simulink model "mppt_solar"  (R2024b)
settings: Solver=VariableStepAuto  StartTime=0.0  StopTime=1  RelTol=1e-3
libraries: spsSeriesRLCBranchLib x4, spsDiodeLib x2, spsCurrentMeasurementLib x1, spsMosfetLib x1, spsPVArrayLib x1, spsPWMGeneratorDCDCLib x1, spsVoltageMeasurementLib x1, spspowerguiLib x1
settings Model: Creator=saaka  LastModifiedBy=Ram
settings ModelReferenceCC: EnableRefExpFcnMdlSchedulingChecks=on
settings RTWCC: GPUComputeCapability=3.5

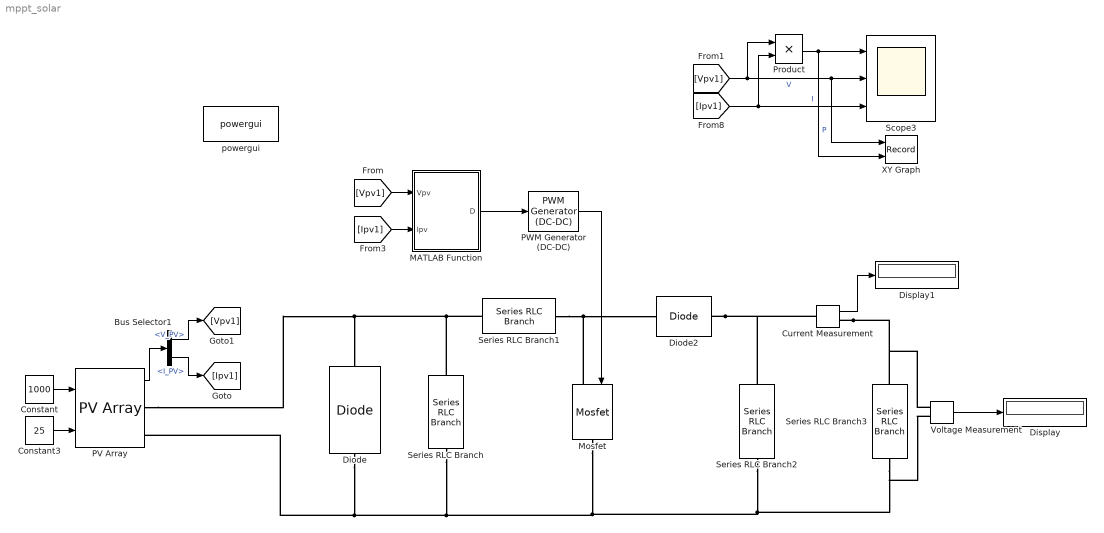
== system mppt_solar ==
  Bus Selector1 : BusSelector  OutputSignals=V_PV,I_PV
  Constant : Constant  Value=1000
  Constant3 : Constant  Value=25
  Current Measurement : spsCurrentMeasurementLib/Current Measurement  PhasorSimulation=off  OutputType=Complex  PSBequivalent=0
  Diode : spsDiodeLib/Diode  Ron=0.001  Lon=0  Vf=0.8  IC=0  UseSnubber=0  Rs=500  Cs=250e-9  Measurements=off
  Diode2 : spsDiodeLib/Diode  Ron=0.001  Lon=0  Vf=0.8  IC=0  UseSnubber=0  Rs=500  Cs=250e-9  Measurements=off
  Display : Display
  Display1 : Display
  MATLAB Function : MATLAB Function  TreatAsAtomicUnit=on
  Mosfet : spsMosfetLib/Mosfet  Ron=0.1  Lon=0  Rd=0.01  Vfd=0  IC=0  Rs=1e5  Cs=inf  Measurements=off
  PV Array : spsPVArrayLib/PV Array  Npar=1  Nser=1  PlotType=array @ 1000 W/m2 & specified temperatures  S_vec="[ 1000  500  100 ]"  Temp_C_vec="[ 45 25  ]"  ModuleName=User-defined  PlotWhenSelected=off  Pm=40.04  Ncell=36  Voc=22.5  Isc=2.22  Vm=19.25  Im=2.08  beta_Voc_pc=-0.36099  alpha_Isc_pc=0.102  beta_Voc=-0.081223  alpha_Isc=0.0022644  IL=2.2218  I0=8.2538e-11  nI=1.0138  Rsh=483.6839  Rs=0.18035  RobustModel=off  RobustCellTemperature=313.3991  BAL=on  Tc=1e-6  Tfilter=5e-5
  PWM Generator (DC-DC) : spsPWMGeneratorDCDCLib/PWM Generator (DC-DC)  Fsw=5000  Ts=0
  Product : Product
  Scope3 : Scope  NumInputPorts=3
  Series RLC Branch : spsSeriesRLCBranchLib/Series RLC Branch  LConnTagsString=__new0  RConnTagsString=__new0  BranchType=C  Resistance=1  Inductance=1e-3  SetiL0=off  InitialCurrent=0  Capacitance=300e-6  Setx0=off  InitialVoltage=0  Measurements=None
  Series RLC Branch1 : spsSeriesRLCBranchLib/Series RLC Branch  LConnTagsString=__new0  RConnTagsString=__new0  BranchType=L  Resistance=1  Inductance=2e-3  SetiL0=off  InitialCurrent=0  Capacitance=1e-6  Setx0=off  InitialVoltage=0  Measurements=None
  Series RLC Branch2 : spsSeriesRLCBranchLib/Series RLC Branch  LConnTagsString=__new0  RConnTagsString=__new0  BranchType=C  Resistance=1  Inductance=1e-3  SetiL0=off  InitialCurrent=0  Capacitance=220e-6  Setx0=off  InitialVoltage=0  Measurements=None
  Series RLC Branch3 : spsSeriesRLCBranchLib/Series RLC Branch  LConnTagsString=__new0  RConnTagsString=__new0  BranchType=R  Resistance=20  Inductance=1e-3  SetiL0=off  InitialCurrent=0  Capacitance=1e-6  Setx0=off  InitialVoltage=0  Measurements=None
  Voltage Measurement : spsVoltageMeasurementLib/Voltage Measurement  PhasorSimulation=off  OutputType=Complex  PSBequivalent=0
  XY Graph : Record  FileSettingsInternal="{\"entries\":[{\"content\":{\"excelSettings\":{\"content\":{},\"type\":\"Streamout.ExcelSettings\"}},\"type\":\"Streamout.FileSettingStorage\",\"uuid\":\"\"}],\"packageUris\":[\"http:\\/\\/schema.mathworks.com\\/mf0\\/streamout_blocks\\/R2020a\"],\"version\":\"1.0\"}"  Layout=[1 1]  SignalsInternal="{\"entries\":[{\"content\":{\"signals\":[{\"content\":{\"blockPath\":[],\"dimensions\":[1],\"domain\":\"\",\"lineColor\":\"#a2142f\",\"plots\":[ 1 ],\"port\":1,\"sid\":[\"\"],\"signalID\":1,\"signalName\":\"V\"},\"type\":\"RecordBlkView.Signal\",\"uuid\":\"\"},{\"content\":{\"blockPath\":[],\"dimensions\":[1],\"domain\":\"\",\"lineColor\":\"#139fff\",\"plots\":[ 1 ],\"port\":2,\"sid\":[\"\"],\"signalID\":2,\"signalName\":\"P\"},\"type\":\"RecordBlkView.Signal\",\"uuid\":\"\"}]},\"type\":\"RecordBlkView.InputSignals\",\"uuid\":\"\"}],\"packageUris\":[\"http:\\/\\/schema.mathworks.com\\/mf0\\/streamout_blocks\\/R2020a\"],\"version\":\"1.0\"}"  VisualizationBindings="{\"xyplotplugin\":{\"info\":[{\"series\":[{\"bindingParametersList\":[{\"parameter\":\"X-Axis\",\"signalID\":1,\"signalName\":\"V\"},{\"parameter\":\"Y-Axis\",\"signalID\":2,\"signalName\":\"P\"},{\"parameter\":\"X-Axis\",\"signalID\":1,\"signalName\":\"V\"},{\"parameter\":\"Y-Axis\",\"signalID\":2,\"signalName\":\"P\"}],\"seriesID\":0}],\"subplotID\":1}]}}"  CompatibilityTag=XY
  powergui : spspowerguiLib/powergui  Priority=1  SimulationMode=Continuous  SampleTime=50e-6  frequency=60  Iterations=50  frequencyindice=0  Pbase=100e6  ErrMax=1e-4  UnitsV=kV  UnitsW=MW  buscounter=0  FunctionMessages=off  echomessages=off  EnableUseOfTLC=off  CurrentSourceSwitches=off  DisableSnubberDevices=off  DisableRonSwitches=off  DisableVfSwitches=off  DisplayEquations=off  AutomaticDiscreteSolvers=off  SolverType=Tustin/Backward Euler (TBE)  Interpol=off  ExternalGateDelay=off  methode=off  Ts=100  x0status=blocks  SPID=on  SwTol=0  HookPort=off  NonlinearTolerance=1e-4  nMaxIteration=100  ContinueOnMaxIteration=off  RestoreLinks=warning  ResistiveCurrentMeasurement=off  Frange=[0:2:500]  Ylog=off  Xlog=on  ShowGrid=off  save=off  variable=ZData  structure=0  ZoomFFT=off  StartTime=0.0  cycles=1  DisplayStyle=1  fundamental=60  FreqAxis=off  MaxFrequency=1000  frequencyindicesteady=1  RmsSteady=1  display=off
  wires:
  Constant/1 -> PV Array/1
  Constant3/1 -> PV Array/2
  Current Measurement/1 -> Display1/1
  Voltage Measurement/1 -> Display/1
  [Vpv1] -> MATLAB Function/1(Vpv)
  [Ipv1] -> MATLAB Function/2(Ipv)
  MATLAB Function/1(D) -> PWM Generator (DC-DC)/1
  PWM Generator (DC-DC)/1 -> Mosfet/1
  PV Array/1 -> Bus Selector1/1
  Bus Selector1/2 -> [Ipv1]  "<I_PV>"
  Bus Selector1/1 -> [Vpv1]  "<V_PV>"
  [Vpv1] -> Product/1, XY Graph/1, Scope3/2  "V"
  [Ipv1] -> Product/2, Scope3/3  "I"
  Product/1 -> XY Graph/2, Scope3/1  "P"
  connections:
  Voltage Measurement/LConn2 -- Series RLC Branch3/RConn1 -- Series RLC Branch2/RConn1 -- Mosfet/RConn1 -- Diode/LConn1 -- PV Array/RConn2 -- Series RLC Branch/RConn1
  Current Measurement/RConn1 -- Series RLC Branch3/LConn1 -- Voltage Measurement/LConn1
  Diode2/RConn1 -- Series RLC Branch2/LConn1 -- Current Measurement/LConn1
  Series RLC Branch/LConn1 -- PV Array/RConn1 -- Diode/RConn1 -- Series RLC Branch1/LConn1
  Series RLC Branch1/RConn1 -- Mosfet/LConn1 -- Diode2/LConn1

== matlab function mppt_solar/MATLAB Function ==
  settings: updateMethod=DISCRETE
  data: Vpv input; D output; Ipv input
function D = PandO(Vpv,Ipv)
persistent Dprev Pprev Vprev
if isempty(Dprev)
    Dprev=0.7;
    Vprev=190;
    Pprev=2000;
end
deltaD=0.001;
Ppv=Vpv*Ipv;
if (Ppv-Pprev)~=0
    if(Ppv-Pprev)>0
        if(Vpv-Vprev)>0
            D=Dprev-deltaD;
        else
            D=Dprev+deltaD;
        end
    else
        if(Vpv-Vprev)>0
            D=Dprev+deltaD;
        else
            D=Dprev-deltaD;
        end
    end
else
    D=Dprev;
end

Dprev=D;
Vprev=Vpv;
Pprev=Ppv;
